simulink model "LF_Week2_OpenLoop"  (R2025b)
settings: Solver=FixedStepDiscrete  StartTime=0.0  StopTime=cfg.stop_time  FixedStep=cfg.Ts  RelTol=1e-3
model workspace (MAT data in the model file):
  Kd = 0.03
  Kp = 0.45
  cfg.root = 'F:\DIGITAL TWEEN\line_follower_twin\weeks1_4'
  cfg.trackMask = [0 0 0 0 0 0 0 0 0 0 0 0 ... (276271 elements, 431x641)]
  cfg.trackReflectance = [0 0 0 0 0 0 0 0 0 0 0 0 ... (276271 elements, 431x641)]
  cfg.map_width_m = 2.56
  cfg.map_height_m = 1.72
  cfg.meters_per_pixel_x = 0.004
  cfg.meters_per_pixel_y = 0.004
  cfg.line_width_m = 0.02
  cfg.stroke_width_px = 5
  cfg.referenceXY = [0.48 0.484 0.488 0.492 0.496 0.5 0.504 0.508 0.512 0.516 0.52 0.524 ... (6258 elements, 3129x2)]
  cfg.referenceArc = [0 0.004 0.008 0.012 0.016 0.02 0.024 0.028 0.032 0.036 0.04 0.044 ... (3129 elements, 1x3129)]
  cfg.x0 = 0.48
  cfg.y0 = 0.196
  cfg.theta0 = 0
  cfg.Ts = 0.02
  cfg.wheel_base_m = 0.12
  cfg.body_length_m = 0.16
  cfg.body_width_m = 0.1
  cfg.sensor_front_m = 0.05
  cfg.sensor_spacing_m = 0.008
  cfg.sensor_weights = [3.5 2.5 1.5 0.5 -0.5 -1.5 -2.5 -3.5]
  cfg.km = 0.35
  cfg.base_speed = 0.35
  cfg.Kp = 0.45
  cfg.Kd = 0.03
  cfg.Ki = 0
  cfg.derivative_tau = 0.08
  cfg.sensor_threshold = 0.5
  cfg.loss_timeout_s = 0.2
  cfg.stop_time = 100
  cfg.results_dir = 'F:\DIGITAL TWEEN\line_follower_twin\weeks1_4\results'
  cfg.models_dir = 'F:\DIGITAL TWEEN\line_follower_twin\weeks1_4\models'
  uL = 0.5
  uR = 0.5
undefined symbols (not defined in the file): DiscIntNeverNeededParam
settings Model: Creator=Xiaol  LastModifiedBy=Xiaol
settings DataIOCC: SaveOutput=off  SignalLogging=off

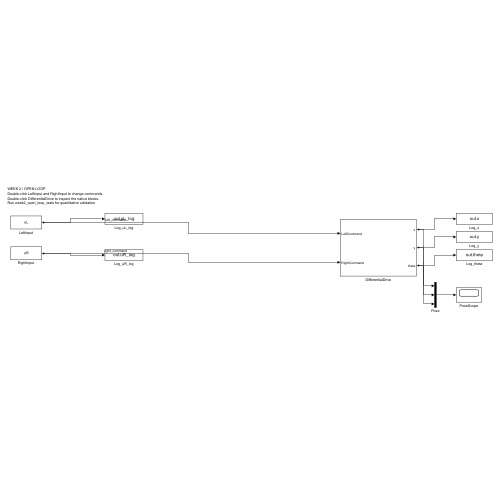
[thumbnail: Simulink's stored preview of the top-level diagram]
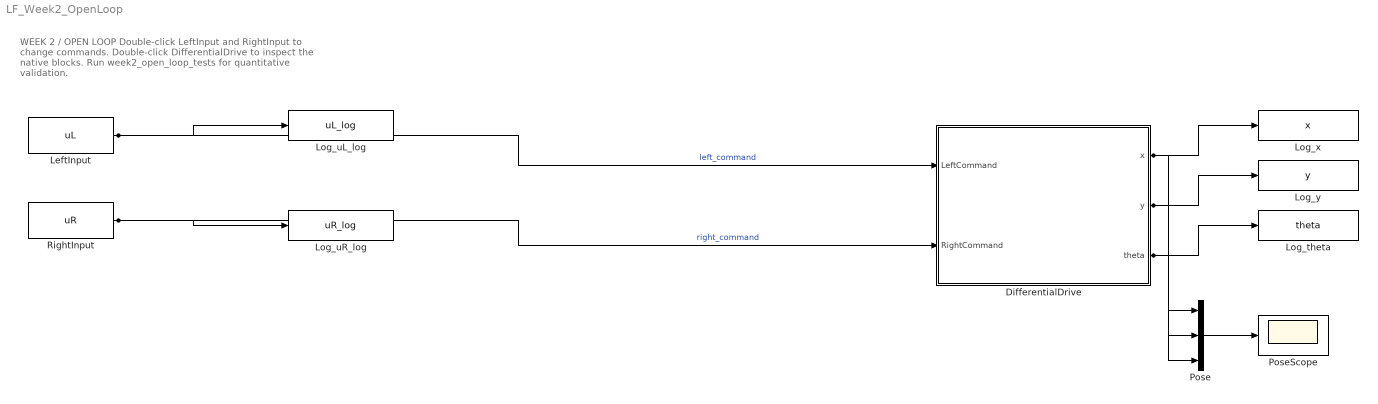
== system LF_Week2_OpenLoop ==
  note: WEEK 2 / OPEN LOOP
      | Double-click LeftInput and RightInput to change commands.
      | Double-click DifferentialDrive to inspect the native blocks.
      | Run week2_open_loop_tests for quantitative validation.
  DifferentialDrive : Subsystem
  LeftInput : Constant  Value=uL  SampleTime=cfg.Ts
  Log_theta : ToWorkspace  VariableName=theta  SaveFormat=Timeseries  SampleTime=-1
  Log_uL_log : ToWorkspace  VariableName=uL_log  SaveFormat=Timeseries  SampleTime=-1
  Log_uR_log : ToWorkspace  VariableName=uR_log  SaveFormat=Timeseries  SampleTime=-1
  Log_x : ToWorkspace  VariableName=x  SaveFormat=Timeseries  SampleTime=-1
  Log_y : ToWorkspace  VariableName=y  SaveFormat=Timeseries  SampleTime=-1
  Pose : Mux  Inputs=3
  PoseScope : Scope
  RightInput : Constant  Value=uR  SampleTime=cfg.Ts
  wires:
  DifferentialDrive/1(x) -> Log_x/1, Pose/1
  DifferentialDrive/2(y) -> Log_y/1, Pose/2
  DifferentialDrive/3(theta) -> Log_theta/1, Pose/3
  Pose/1 -> PoseScope/1
  LeftInput/1 -> DifferentialDrive/1(LeftCommand), Log_uL_log/1  "left_command"
  RightInput/1 -> DifferentialDrive/2(RightCommand), Log_uR_log/1  "right_command"

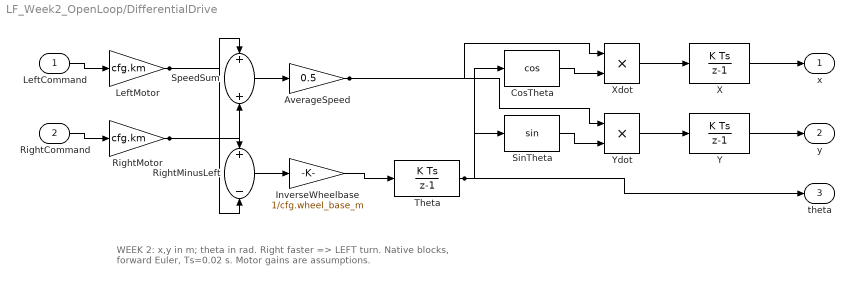
== system LF_Week2_OpenLoop/DifferentialDrive ==
  note: WEEK 2: x,y in m; theta in rad. Right faster => LEFT turn.
      | Native blocks, forward Euler, Ts=0.02 s. Motor gains are assumptions.
  LeftCommand : Inport
  RightCommand : Inport  Port=2
  AverageSpeed : Gain  Gain=0.5
  CosTheta : Trigonometry  Operator=cos
  InverseWheelbase : Gain  Gain=1/cfg.wheel_base_m
  LeftMotor : Gain  Gain=cfg.km
  RightMinusLeft : Sum  Inputs=+-
  RightMotor : Gain  Gain=cfg.km
  SinTheta : Trigonometry
  SpeedSum : Sum
  Theta : DiscreteIntegrator  gainval=1  InitialCondition=cfg.theta0  SampleTime=cfg.Ts  ICPrevOutput=DiscIntNeverNeededParam  ICPrevScaledInput=DiscIntNeverNeededParam
  X : DiscreteIntegrator  gainval=1  InitialCondition=cfg.x0  SampleTime=cfg.Ts  ICPrevOutput=DiscIntNeverNeededParam  ICPrevScaledInput=DiscIntNeverNeededParam
  Xdot : Product
  Y : DiscreteIntegrator  gainval=1  InitialCondition=cfg.y0  SampleTime=cfg.Ts  ICPrevOutput=DiscIntNeverNeededParam  ICPrevScaledInput=DiscIntNeverNeededParam
  Ydot : Product
  x : Outport
  y : Outport  Port=2
  theta : Outport  Port=3
  wires:
  LeftCommand/1 -> LeftMotor/1
  RightCommand/1 -> RightMotor/1
  LeftMotor/1 -> SpeedSum/1, RightMinusLeft/2
  RightMotor/1 -> SpeedSum/2, RightMinusLeft/1
  SpeedSum/1 -> AverageSpeed/1
  RightMinusLeft/1 -> InverseWheelbase/1
  InverseWheelbase/1 -> Theta/1
  Theta/1 -> CosTheta/1, SinTheta/1, theta/1
  AverageSpeed/1 -> Xdot/1, Ydot/1
  CosTheta/1 -> Xdot/2
  SinTheta/1 -> Ydot/2
  Xdot/1 -> X/1
  Ydot/1 -> Y/1
  X/1 -> x/1
  Y/1 -> y/1
